simulink model "PerceptionAndControl"  (R2026b)
settings: Solver=FixedStepAuto  StopTime=TFinal
settings Model: Creator=The MathWorks, Inc.  LastModifiedBy=The MathWorks, Inc.
settings SolverCC: PositivePriorityOrder=on
settings OptimizationCC: DifferentSizesBufferReuse=on  EfficientTunableParamExpr=on  EnhancedBackFolding=on  MaxStackSize=64  OptimizationCustomize=off  OptimizeBlockOrder=speed  PassReuseOutputArgsAs=Individual arguments  RemoveInternalMemoryZeroInit=on  RemoveRootLevelIOMemoryZeroInit=on
settings DebuggingCC: ParameterTunabilityLossMsg=error
settings HardwareCC: ProdHWDeviceType=ARM Compatible->ARM Cortex  ProdLargestAtomicFloat=Double  ProdLargestAtomicInteger=Long  ProdLongLongMode=on
settings SFSimCC: MATLABDynamicMemAlloc=off  SimTargetLang=C++
settings RTWCC: Description=Embedded Coder  HardwareBoard=PX4 Pixhawk 6c  SystemTargetFile=ert.tlc  TLCOptions="-aInlineSetEventsForThisBaseRateFcn=TLC_FALSE -aSuppressMultiTaskScheduler=TLC_FALSE  -aRateBasedStepFcn=0"  TargetLang=C++  TemplateMakefile=ert_default_tmf  Toolchain=GNU Tools for PX4 Autopilots
settings CodeAppCC: ForceParamTrailComments=on  IgnoreCustomStorageClasses=off  InsertBlockDesc=on  OperatorAnnotations=on  SFDataObjDesc=on  SimulinkDataObjDesc=on
settings ERTTargetCC: ExtModeIntrfLevel=Level2 - Open  ExtModeMexFile=ext_xcp  ExtModeStaticAlloc=on

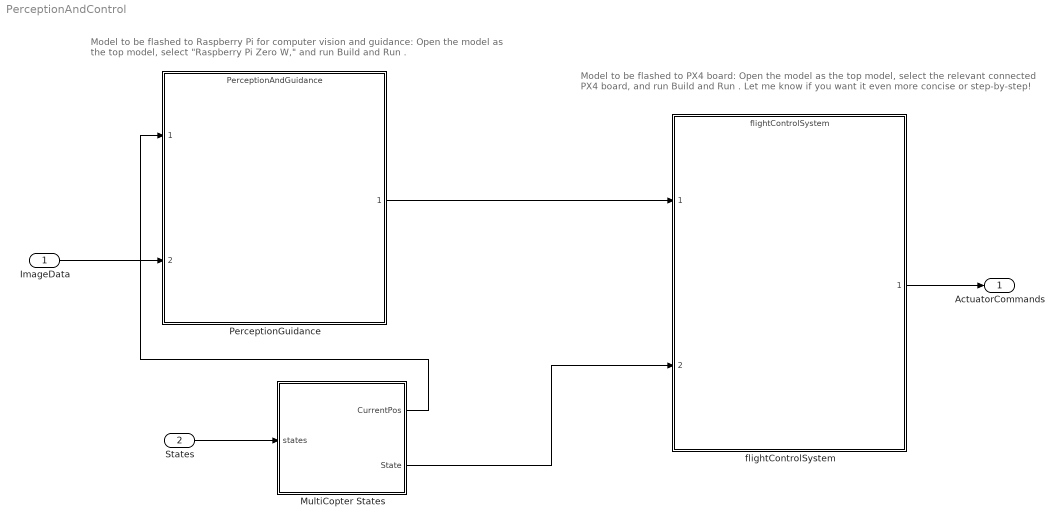
== system PerceptionAndControl ==
  note: Model to be flashed to Raspberry Pi for computer vision and guidance:
      | Open the model as the top model, select "Raspberry Pi Zero W," and run Build and Run .
  note: Model to be flashed to PX4 board:
      | Open the model as the top model, select the relevant connected PX4 board, and run Build and Run .
      | Let me know if you want it even more concise or step-by-step!
  ImageData : Inport  OutDataTypeStr=uint8  PortDimensions=[120, 160, 3]
  States : Inport  Port=2  OutDataTypeStr=Bus: UAVStatesBus
  MultiCopter States : Subsystem  Variant=on
  PerceptionGuidance : ModelReference  ModelNameDialog=PerceptionAndGuidance.slx  SimulationMode=Normal  ModelReferenceVersion=7.96
  flightControlSystem : ModelReference  ModelNameDialog=flightControlSystem.slx  SimulationMode=Normal  ModelReferenceVersion=11.61
  ActuatorCommands : Outport  OutDataTypeStr=Bus: setPWMInput
  wires:
  flightControlSystem/1 -> ActuatorCommands/1
  PerceptionGuidance/1 -> flightControlSystem/1
  ImageData/1 -> PerceptionGuidance/2
  MultiCopter States/1(CurrentPos) -> PerceptionGuidance/1
  MultiCopter States/2(State) -> flightControlSystem/2
  States/1 -> MultiCopter States/1(states)

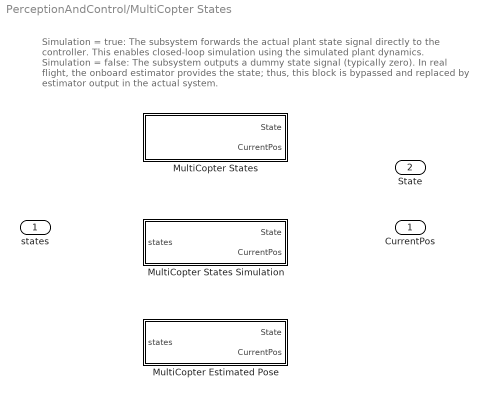
== system PerceptionAndControl/MultiCopter States ==
  note: Simulation = true:
      | The subsystem forwards the actual plant state signal directly to the controller. This enables closed-loop simulation using the simulated plant dynamics.
      |
      | Simulation = false:
      | The subsystem outputs a dummy state signal (typically zero). In real flight, the onboard estimator provides the state; thus, this block is bypassed and replaced by estimator output in the actual system.
  states : Inport
  MultiCopter Estimated Pose : Subsystem  VariantControl=(Simulation == false && CompanionComputer == false)
  MultiCopter States : Subsystem  VariantControl=(Simulation == false && CompanionComputer == true)
  MultiCopter States Simulation : Subsystem  VariantControl=Simulation == true
  CurrentPos : Outport
  State : Outport  Port=2

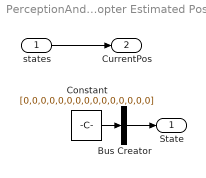
== system PerceptionAndControl/MultiCopter States/MultiCopter Estimated Pose ==
  states : Inport
  Bus Creator : BusCreator  Inputs=1  OutDataTypeStr=Bus: UAVStatesBus
  Constant : Constant  Value=[0,0,0,0,0,0,0,0,0,0,0,0,0,0,0]  SampleTime=-1
  State : Outport
  CurrentPos : Outport  Port=2
  wires:
  Constant/1 -> Bus Creator/1
  Bus Creator/1 -> State/1
  states/1 -> CurrentPos/1

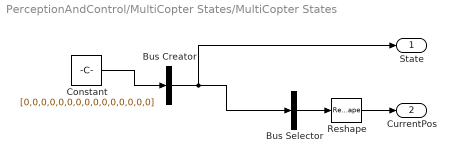
== system PerceptionAndControl/MultiCopter States/MultiCopter States ==
  Bus Creator : BusCreator  Inputs=1  OutDataTypeStr=Bus: UAVStatesBus
  Bus Selector : BusSelector  OutputSignals=X,Y,Z,yaw  OutputAsBus=on
  Constant : Constant  Value=[0,0,0,0,0,0,0,0,0,0,0,0,0,0,0]  SampleTime=-1
  Reshape : Reshape
  State : Outport
  CurrentPos : Outport  Port=2
  wires:
  Bus Selector/1 -> Reshape/1
  Reshape/1 -> CurrentPos/1
  Constant/1 -> Bus Creator/1
  Bus Creator/1 -> State/1, Bus Selector/1

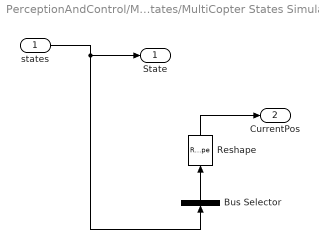
== system PerceptionAndControl/MultiCopter States/MultiCopter States Simulation ==
  states : Inport
  Bus Selector : BusSelector  OutputSignals=X,Y,Z,yaw  OutputAsBus=on
  Reshape : Reshape
  State : Outport
  CurrentPos : Outport  Port=2
  wires:
  Bus Selector/1 -> Reshape/1
  states/1 -> State/1, Bus Selector/1
  Reshape/1 -> CurrentPos/1
